simulink model "Sistemap2"  (R2026a)
settings: Solver=ode15s  StopTime=15  MaxStep=1E-2
libraries: fl_lib x7, nesl_utility x3, slpidlib x2
settings Model: Creator=Admin  LastModifiedBy=HP
settings DataIOCC: TimeSaveName=t
settings DebuggingCC: ArtificialAlgebraicLoopMsg=none  MaxConsecutiveZCsMsg=none

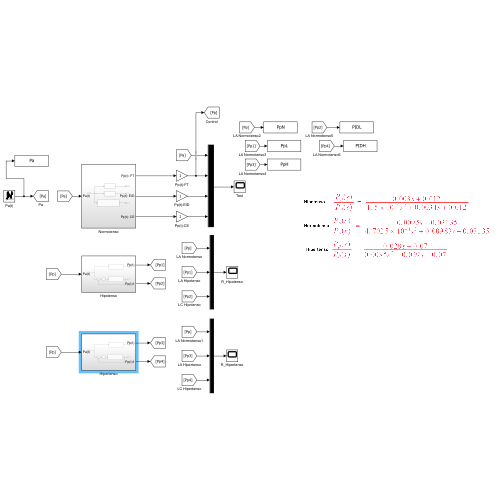
[thumbnail: Simulink's stored preview of the top-level diagram]
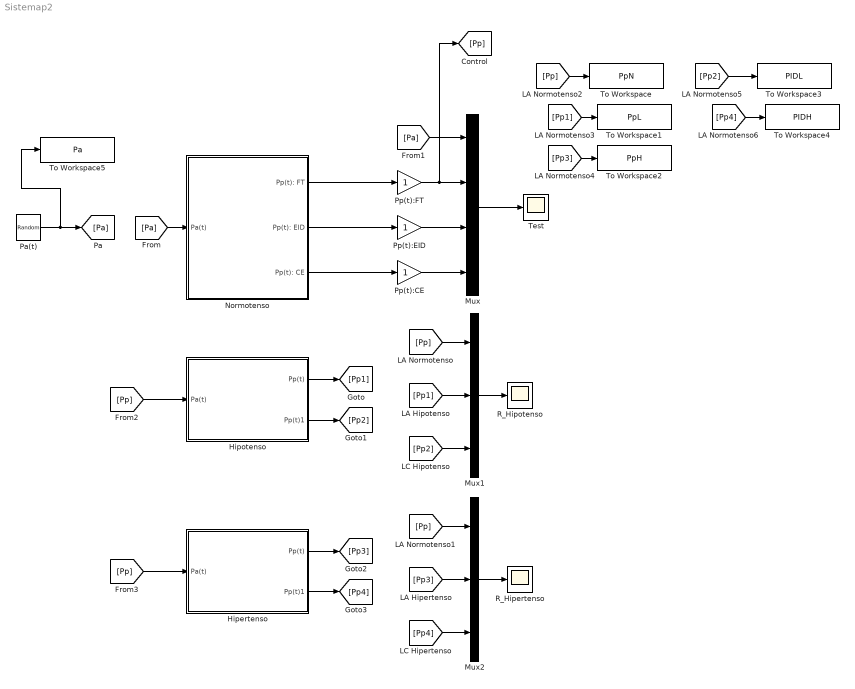
== system Sistemap2 ==
  Hipertenso : Subsystem
  Hipotenso : Subsystem
  Mux : Mux
  Mux1 : Mux  Inputs=3
  Mux2 : Mux  Inputs=3
  Normotenso : Subsystem
  Pa(t) : UniformRandomNumber  Minimum=-0.2  Seed=106  SampleTime=0.1
  Pp(t):CE : Gain
  Pp(t):EID : Gain
  Pp(t):FT : Gain
  R_Hipertenso : Scope
      settings: ActiveDisplayYMinimum=-0.4  ActiveDisplayYMaximum=1.2  DataLoggingVariableName=ScopeData2
  R_Hipotenso : Scope
      settings: ActiveDisplayYMinimum=-0.4  ActiveDisplayYMaximum=1.2
  Test : Scope
      settings: TimeSpan=10  ActiveDisplayYMinimum=-0.21660297738034551  ActiveDisplayYMaximum=1.0433970226196547
  To Workspace : ToWorkspace  VariableName=PpN  SampleTime=-1
  To Workspace1 : ToWorkspace  VariableName=PpL  SampleTime=-1
  To Workspace2 : ToWorkspace  VariableName=PpH  SampleTime=-1
  To Workspace3 : ToWorkspace  VariableName=PIDL  SampleTime=-1
  To Workspace4 : ToWorkspace  VariableName=PIDH  SampleTime=-1
  To Workspace5 : ToWorkspace  VariableName=Pa  SampleTime=-1
  wires:
  [Pa] -> Normotenso/1(Pa(t))
  Pa(t)/1 -> To Workspace5/1, [Pa]
  Normotenso/3(Pp(t): CE) -> Pp(t):CE/1
  Normotenso/2(Pp(t): EID) -> Pp(t):EID/1
  Normotenso/1(Pp(t): FT) -> Pp(t):FT/1
  [Pa] -> Mux/1
  Mux/1 -> Test/1
  Pp(t):FT/1 -> [Pp], Mux/2
  Pp(t):EID/1 -> Mux/3
  Pp(t):CE/1 -> Mux/4
  [Pp] -> Hipotenso/1(Pa(t))
  [Pp] -> Mux1/1
  [Pp1] -> Mux1/2
  [Pp2] -> Mux1/3
  Mux1/1 -> R_Hipotenso/1
  Hipotenso/1(Pp(t)) -> [Pp1]
  Hipotenso/2(Pp(t)1) -> [Pp2]
  [Pp] -> Hipertenso/1(Pa(t))
  Mux2/1 -> R_Hipertenso/1
  [Pp4] -> Mux2/3
  [Pp3] -> Mux2/2
  [Pp] -> Mux2/1
  Hipertenso/1(Pp(t)) -> [Pp3]
  Hipertenso/2(Pp(t)1) -> [Pp4]
  [Pp] -> To Workspace/1
  [Pp1] -> To Workspace1/1
  [Pp3] -> To Workspace2/1
  [Pp4] -> To Workspace4/1
  [Pp2] -> To Workspace3/1

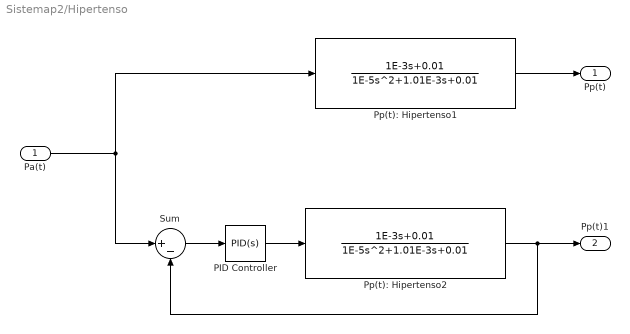
== system Sistemap2/Hipertenso ==
  Pa(t) : Inport
  PID Controller : slpidlib/PID Controller  Controller=PID  Form=Parallel  TimeDomain=Continuous-time  UseExternalTs=off  SampleTime=-1  IntegratorMethod=Forward Euler  FilterMethod=Forward Euler  ControllerParametersSource=internal  P=10.6371299938513  I=3103.214314844  UseKiTs=off  D=0.00184067808796981  UseExternalDerivativeSource=off  N=3062.3767896367  UseFilter=on  TunerSelectOption=Transfer Function Based (PID Tuner App)  InitialConditionSource=internal  InitialConditionForIntegrator=0  InitialConditionForFilter=0  DifferentiatorICPrevScaledInput=0  ExternalReset=none  TrackingMode=off  Kt=1  LimitOutput=off  SatLimitsSource=internal  UpperSaturationLimit=inf  LowerSaturationLimit=-inf  LinearizeAsGain=on  AntiWindupMode=none  Kb=1  LimitIntegrator=off  UpperIntegratorSaturationLimit=inf  LowerIntegratorSaturationLimit=-inf  POutMin=[]  POutMax=[]  IOutMin=[]  IOutMax=[]  DOutMin=[]  DOutMax=[]  NOutMin=[]  NOutMax=[]  SumOutMin=[]  SumOutMax=[]  SaturationOutMin=[]  SaturationOutMax=[]  PParamMin=[]  PParamMax=[]  IParamMin=[]  IParamMax=[]  DParamMin=[]  DParamMax=[]  NParamMin=[]  NParamMax=[]  KbParamMin=[]  KbParamMax=[]  KtParamMin=[]  KtParamMax=[]  KbOutMin=[]  KbOutMax=[]  KtOutMin=[]  KtOutMax=[]  IntegratorOutMin=[]  IntegratorOutMax=[]  FilterOutMin=[]  FilterOutMax=[]  SumI1OutMin=[]  SumI1OutMax=[]  SumI2OutMin=[]  SumI2OutMax=[]  SumI3OutMin=[]  SumI3OutMax=[]  SumI4OutMin=[]  SumI4OutMax=[]  SumDOutMin=[]  SumDOutMax=[]  DifferentiatorOutMin=[]  DifferentiatorOutMax=[]  FilterDiffOutCoefMin=[]  FilterDiffOutCoefMax=[]  ReciprocalOutMin=[]  ReciprocalOutMax=[]  SumDenOutMin=[]  SumDenOutMax=[]  SumNumOutMin=[]  SumNumOutMax=[]  DivideOutMin=[]  DivideOutMax=[]  UdiffTsProdOutMin=[]  UdiffTsProdOutMax=[]  NTsProdOutMin=[]  NTsProdOutMax=[]  UintegralTsProdOutMin=[]  UintegralTsProdOutMax=[]  UngainTsProdOutMin=[]  UngainTsProdOutMax=[]  ClampingZeroOutDataTypeStr=Inherit: Inherit via back propagation  ClampingZeroOutMin=[]  ClampingZeroOutMax=[]  FilterDenConstantOutDataTypeStr=Inherit: Inherit via back propagation  FilterDenConstantOutMin=[]  FilterDenConstantOutMax=[]  PCopyOutDataTypeStr=Inherit: Inherit via back propagation  PCopyOutMin=[]  PCopyOutMax=[]  NCopyOutDataTypeStr=Inherit: Inherit via back propagation  NCopyOutMin=[]  NCopyOutMax=[]  IntegratorContinuousStateAttributes=''  IntegratorStateMustResolveToSignalObject=off  IntegratorRTWStateStorageClass=Auto  FilterContinuousStateAttributes=''  FilterStateMustResolveToSignalObject=off  FilterRTWStateStorageClass=Auto  ParallelPVariant=InternalParameters  IdealPVariant=Disabled  IVariant=InternalParameters  DVariant=InternalParameters  IntegratorVariant=Continuous  SatVariant=Disabled  AWVariant=Passthrough  PCopyVariant=Disabled  TRVariant=Disabled  FdbkBlocksVariant=Forward  IdealPFdbkVariant=Disabled  SatFdbkVariant=Disabled  DerivativeFilterVariant=ContFilter  NVariant=InternalParameters  NCopyVariant=Disabled  FilterICVariant=InternalICsFilter  IntegratorICVariant=InternalICs  ExternalResetVariant=Disabled  TRSumVariant=Passthrough  SumFdbkVariant=Disabled  SumVariant=Sum_PID  TsampFilterVariant=InternalTs  TsampNgainVariant=Passthrough  TsampIntegralVariant=Disabled_SignalSpec  ExternalSaturationOutDataTypeStr=Inherit: Same as second input  DerivativeSourceVariant=ErrorSignal  PreIntVariant=InternalPreInt
  Pp(t): Hipertenso1 : TransferFcn  Numerator=[1E-3,0.01]  Denominator=[1E-5, 1.01E-3, 0.01]
  Pp(t): Hipertenso2 : TransferFcn  Numerator=[1E-3,0.01]  Denominator=[1E-5, 1.01E-3, 0.01]
  Sum : Sum  Inputs=|+-
  Pp(t) : Outport
  Pp(t)1 : Outport  Port=2
  wires:
  Pp(t): Hipertenso1/1 -> Pp(t)/1
  Sum/1 -> PID Controller/1
  Pa(t)/1 -> Pp(t): Hipertenso1/1, Sum/1
  PID Controller/1 -> Pp(t): Hipertenso2/1
  Pp(t): Hipertenso2/1 -> Sum/2, Pp(t)1/1

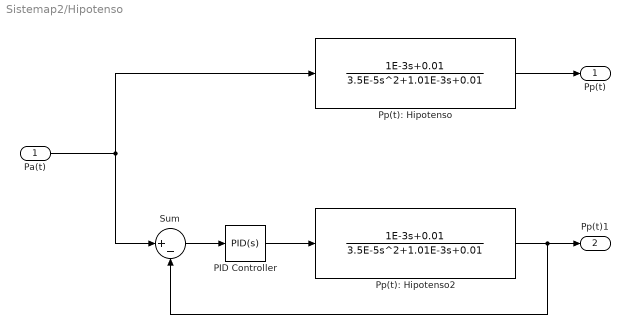
== system Sistemap2/Hipotenso ==
  Pa(t) : Inport
  PID Controller : slpidlib/PID Controller  Controller=PID  Form=Parallel  TimeDomain=Continuous-time  UseExternalTs=off  SampleTime=-1  IntegratorMethod=Forward Euler  FilterMethod=Forward Euler  ControllerParametersSource=internal  P=45.9868123888852  I=11182.6730763462  UseKiTs=off  D=0.00586447466175754  UseExternalDerivativeSource=off  N=5005.76250783319  UseFilter=on  TunerSelectOption=Transfer Function Based (PID Tuner App)  InitialConditionSource=internal  InitialConditionForIntegrator=0  InitialConditionForFilter=0  DifferentiatorICPrevScaledInput=0  ExternalReset=none  TrackingMode=off  Kt=1  LimitOutput=off  SatLimitsSource=internal  UpperSaturationLimit=inf  LowerSaturationLimit=-inf  LinearizeAsGain=on  AntiWindupMode=none  Kb=1  LimitIntegrator=off  UpperIntegratorSaturationLimit=inf  LowerIntegratorSaturationLimit=-inf  POutMin=[]  POutMax=[]  IOutMin=[]  IOutMax=[]  DOutMin=[]  DOutMax=[]  NOutMin=[]  NOutMax=[]  SumOutMin=[]  SumOutMax=[]  SaturationOutMin=[]  SaturationOutMax=[]  PParamMin=[]  PParamMax=[]  IParamMin=[]  IParamMax=[]  DParamMin=[]  DParamMax=[]  NParamMin=[]  NParamMax=[]  KbParamMin=[]  KbParamMax=[]  KtParamMin=[]  KtParamMax=[]  KbOutMin=[]  KbOutMax=[]  KtOutMin=[]  KtOutMax=[]  IntegratorOutMin=[]  IntegratorOutMax=[]  FilterOutMin=[]  FilterOutMax=[]  SumI1OutMin=[]  SumI1OutMax=[]  SumI2OutMin=[]  SumI2OutMax=[]  SumI3OutMin=[]  SumI3OutMax=[]  SumI4OutMin=[]  SumI4OutMax=[]  SumDOutMin=[]  SumDOutMax=[]  DifferentiatorOutMin=[]  DifferentiatorOutMax=[]  FilterDiffOutCoefMin=[]  FilterDiffOutCoefMax=[]  ReciprocalOutMin=[]  ReciprocalOutMax=[]  SumDenOutMin=[]  SumDenOutMax=[]  SumNumOutMin=[]  SumNumOutMax=[]  DivideOutMin=[]  DivideOutMax=[]  UdiffTsProdOutMin=[]  UdiffTsProdOutMax=[]  NTsProdOutMin=[]  NTsProdOutMax=[]  UintegralTsProdOutMin=[]  UintegralTsProdOutMax=[]  UngainTsProdOutMin=[]  UngainTsProdOutMax=[]  ClampingZeroOutDataTypeStr=Inherit: Inherit via back propagation  ClampingZeroOutMin=[]  ClampingZeroOutMax=[]  FilterDenConstantOutDataTypeStr=Inherit: Inherit via back propagation  FilterDenConstantOutMin=[]  FilterDenConstantOutMax=[]  PCopyOutDataTypeStr=Inherit: Inherit via back propagation  PCopyOutMin=[]  PCopyOutMax=[]  NCopyOutDataTypeStr=Inherit: Inherit via back propagation  NCopyOutMin=[]  NCopyOutMax=[]  IntegratorContinuousStateAttributes=''  IntegratorStateMustResolveToSignalObject=off  IntegratorRTWStateStorageClass=Auto  FilterContinuousStateAttributes=''  FilterStateMustResolveToSignalObject=off  FilterRTWStateStorageClass=Auto  ParallelPVariant=InternalParameters  IdealPVariant=Disabled  IVariant=InternalParameters  DVariant=InternalParameters  IntegratorVariant=Continuous  SatVariant=Disabled  AWVariant=Passthrough  PCopyVariant=Disabled  TRVariant=Disabled  FdbkBlocksVariant=Forward  IdealPFdbkVariant=Disabled  SatFdbkVariant=Disabled  DerivativeFilterVariant=ContFilter  NVariant=InternalParameters  NCopyVariant=Disabled  FilterICVariant=InternalICsFilter  IntegratorICVariant=InternalICs  ExternalResetVariant=Disabled  TRSumVariant=Passthrough  SumFdbkVariant=Disabled  SumVariant=Sum_PID  TsampFilterVariant=InternalTs  TsampNgainVariant=Passthrough  TsampIntegralVariant=Disabled_SignalSpec  ExternalSaturationOutDataTypeStr=Inherit: Same as second input  DerivativeSourceVariant=ErrorSignal  PreIntVariant=InternalPreInt
  Pp(t): Hipotenso : TransferFcn  Numerator=[1E-3,0.01]  Denominator=[3.5E-5, 1.01E-3, 0.01]
  Pp(t): Hipotenso2 : TransferFcn  Numerator=[1E-3,0.01]  Denominator=[3.5E-5, 1.01E-3, 0.01]
  Sum : Sum  Inputs=|+-
  Pp(t) : Outport
  Pp(t)1 : Outport  Port=2
  wires:
  Pa(t)/1 -> Sum/1, Pp(t): Hipotenso/1
  PID Controller/1 -> Pp(t): Hipotenso2/1
  Sum/1 -> PID Controller/1
  Pp(t): Hipotenso2/1 -> Sum/2, Pp(t)1/1
  Pp(t): Hipotenso/1 -> Pp(t)/1

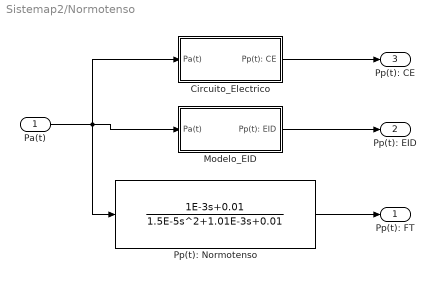
== system Sistemap2/Normotenso ==
  Pa(t) : Inport
  Circuito_Electrico : Subsystem
  Modelo_EID : Subsystem
  Pp(t): Normotenso : TransferFcn  Numerator=[1E-3,0.01]  Denominator=[1.5E-5,1.01E-3,0.01]
  Pp(t): FT : Outport
  Pp(t): EID : Outport  Port=2
  Pp(t): CE : Outport  Port=3
  wires:
  Pa(t)/1 -> Circuito_Electrico/1(Pa(t)), Modelo_EID/1(Pa(t)), Pp(t): Normotenso/1
  Pp(t): Normotenso/1 -> Pp(t): FT/1
  Modelo_EID/1(Pp(t): EID) -> Pp(t): EID/1
  Circuito_Electrico/1(Pp(t): CE) -> Pp(t): CE/1

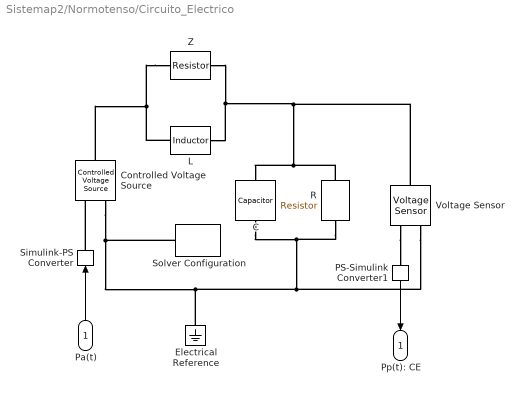
== system Sistemap2/Normotenso/Circuito_Electrico ==
  Pa(t) : Inport
  C : fl_lib/Electrical/Electrical Elements/Capacitor  c=1.500 F  r=1e-6 Ohm  g=0 1/Ohm  i_specify=off  i_priority=None  i=0 A  i_nominal_specify=off  i_nominal_value=1  i_nominal_unit=A  v_specify=off  v_priority=None  v=0 V  v_nominal_specify=off  v_nominal_value=1  v_nominal_unit=V  vc_specify=off  vc_priority=High  vc=0 V  vc_nominal_specify=off  vc_nominal_value=1  vc_nominal_unit=V
  Controlled Voltage Source : fl_lib/Electrical/Electrical Sources/Controlled Voltage Source
  Electrical Reference : fl_lib/Electrical/Electrical Elements/Electrical Reference
  L : fl_lib/Electrical/Electrical Elements/Inductor  l=0.001 H  r=0 Ohm  g=1e-9 1/Ohm  i_specify=off  i_priority=None  i=0 A  i_nominal_specify=off  i_nominal_value=1  i_nominal_unit=A  v_specify=off  v_priority=None  v=0 V  v_nominal_specify=off  v_nominal_value=1  v_nominal_unit=V  i_L_specify=off  i_L_priority=High  i_L=0 A  i_L_nominal_specify=off  i_L_nominal_value=1  i_L_nominal_unit=A
  PS-Simulink Converter1 : nesl_utility/PS-Simulink Converter  PhysicalDomain=network_engine_domain  SubClassName=ps_output  LeftPortType=input  RightPortType=output  PseudoPeriodic=off  Frequencies=[]  VectorFormat=inherit  Unit=inherit  AffineConversion=off
  R : fl_lib/Electrical/Electrical Elements/Resistor  R=1.000 Ohm  i_specify=off  i_priority=None  i=0 A  i_nominal_specify=off  i_nominal_value=1  i_nominal_unit=A  v_specify=off  v_priority=None  v=0 V  v_nominal_specify=off  v_nominal_value=1  v_nominal_unit=V
  Simulink-PS Converter : nesl_utility/Simulink-PS Converter  PhysicalDomain=network_engine_domain  SubClassName=ps_input  LeftPortType=input  RightPortType=output  PseudoPeriodic=off  Frequencies=[]  NoiseDistribution=none  NoiseParameters=[]  Unit=1  AffineConversion=off  FilteringAndDerivatives=provide  SimscapeFilterOrder=1  InputFilterTimeConstant=0.001  UdotUserProvided=0
  Solver Configuration : nesl_utility/Solver Configuration  PhysicalDomain=network_engine_domain  SubClassName=solver  LeftPortType=input  RightPortType=generic  Tones=[]  Harmonics=[]  SimulateNoise=off  Profile=off  UseLocalSampling=off  EnableSwitchedLinearOptims=on  FrequencyDomain=off  UseCCode=off  RelTol=0.001  AbsTol=0.001  MinStep=1e-09  ToWorkspace=off  RevertToSquareIcSolve=off  NumHomotopyIterations=100  PhasorMode=off  PhasorModeNumHarmonics=1  ConsistencySolver=NEWTON_XTOL_AFTER_FTOL  CanonicalOrdering=CANONICAL  OptimizeIntermediates=OPTIMIZED  IndexReductionMethod=DerivativeReplacement  DoDC=off  ResidualTolerance=1e-09  ConsistencyTolSource=GLOBAL  ConsistencyAbsTol=0.001  ConsistencyRelTol=0.001  ConsistencyTolFactor=0.001  UseLocalSolver=off  LocalSolverChoice=NE_BACKWARD_EULER_ADVANCER  ResolveIndetEquations=on  FunctionEvalNumThread=1  LocalSolverSampleTime=0.001  DoFixedCost=off  MaxNonlinIter=3  MaxModeIter=2  ComputeImpulses=off  ImpulseIterations=2  LinearAlgebra=auto  LinearAlgebraNumThread=0  EquationFormulation=NE_TIME_EF  DelaysMemoryBudget=1024  AutomaticFiltering=on  FilteringTimeConstant=0.001  PartitionStorageMethod=AS_NEEDED  PartitionMemoryBudget=1024  PartitionMethod=ROBUST  MultibodyUseLocalSolver=off  MultibodyLocalSolverChoice=ODE1  MultibodyLocalSolverSampleTime=0.001
  Voltage Sensor : fl_lib/Electrical/Electrical Sensors/Voltage Sensor
  Z : fl_lib/Electrical/Electrical Elements/Resistor  R=0.010 Ohm  i_specify=off  i_priority=None  i=0 A  i_nominal_specify=off  i_nominal_value=1  i_nominal_unit=A  v_specify=off  v_priority=None  v=0 V  v_nominal_specify=off  v_nominal_value=1  v_nominal_unit=V
  Pp(t): CE : Outport
  wires:
  PS-Simulink Converter1/1 -> Pp(t): CE/1
  Pa(t)/1 -> Simulink-PS Converter/1
  connections:
  Electrical Reference/LConn1 -- Controlled Voltage Source/RConn2 -- Solver Configuration/RConn1 -- Voltage Sensor/RConn2 -- R/RConn1 -- C/RConn1
  Z/RConn1 -- Controlled Voltage Source/LConn1 -- L/LConn1
  Z/LConn1 -- L/RConn1 -- Voltage Sensor/LConn1 -- R/LConn1 -- C/LConn1
  Voltage Sensor/RConn1 -- PS-Simulink Converter1/LConn1
  Simulink-PS Converter/RConn1 -- Controlled Voltage Source/RConn1

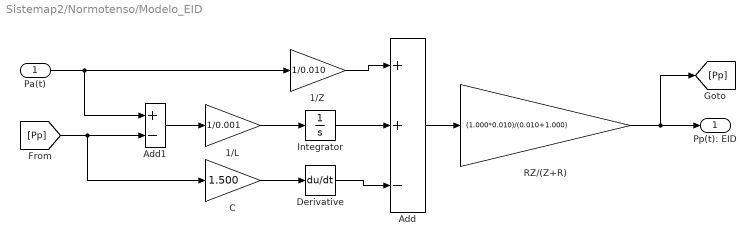
== system Sistemap2/Normotenso/Modelo_EID ==
  Pa(t) : Inport
  1/L : Gain  Gain=1/0.001
  1/Z : Gain  Gain=1/0.010
  Add : Sum  Inputs=++-
  Add1 : Sum  Inputs=+-
  C : Gain  Gain=1.500
  Derivative : Derivative
  Integrator : Integrator
  RZ/(Z+R) : Gain  Gain=(1.000*0.010)/(0.010+1.000)
  Pp(t): EID : Outport
  wires:
  RZ/(Z+R)/1 -> [Pp], Pp(t): EID/1
  1/Z/1 -> Add/1
  Pa(t)/1 -> Add1/1, 1/Z/1
  Add/1 -> RZ/(Z+R)/1
  [Pp] -> C/1, Add1/2
  Add1/1 -> 1/L/1
  1/L/1 -> Integrator/1
  Integrator/1 -> Add/2
  Derivative/1 -> Add/3
  C/1 -> Derivative/1
